simulink model "Actuator_testing"  (R2025b)
settings: Solver=VariableStepAuto  StartTime=0.0  StopTime=10.0  RelTol=1e-3
settings Model: Creator=Admin  LastModifiedBy=Admin

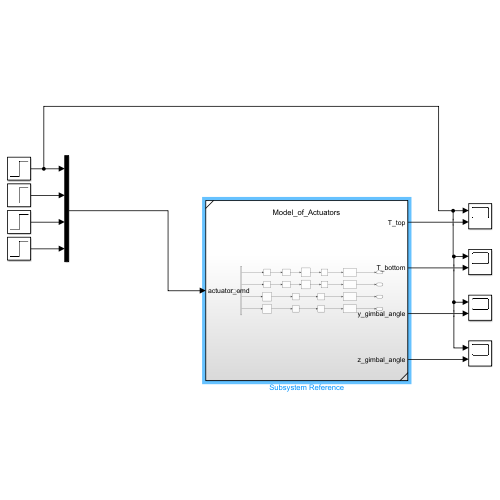
[thumbnail: Simulink's stored preview of the top-level diagram]
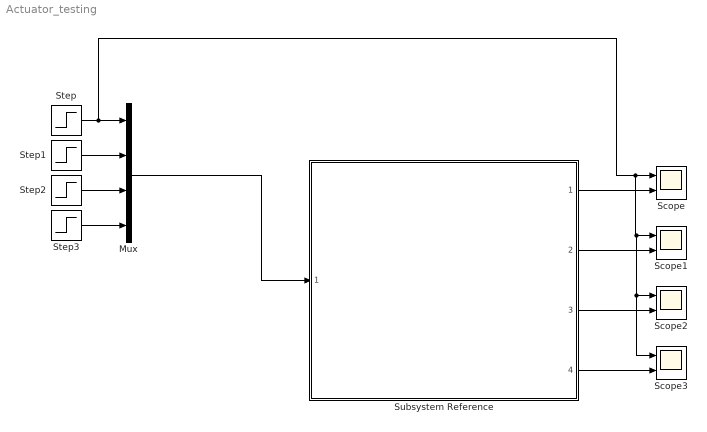
== system Actuator_testing ==
  Mux : Mux
  Scope{,1..3} (4 alike) : Scope  NumInputPorts=2
      Scope settings: ActiveDisplayYMinimum=-0.13072872674571806  ActiveDisplayYMaximum=1.1765585407114627
      Scope1 settings: ActiveDisplayYMinimum=-1  ActiveDisplayYMaximum=1
      Scope2 settings: ActiveDisplayYMinimum=-0.12499999999999997  ActiveDisplayYMaximum=1.125  DataLoggingVariableName=ScopeData2
      Scope3 settings: ActiveDisplayYMinimum=-0.12499999999999997  ActiveDisplayYMaximum=1.125  DataLoggingVariableName=ScopeData3
  Step{,1..3} (4 alike) : Step  SampleTime=0
  Subsystem Reference : Subsystem  ReferencedSubsystem=Model_of_Actuators
  wires:
  Step1/1 -> Mux/2
  Step/1 -> Scope3/1, Scope2/1, Scope1/1, Scope/1, Mux/1
  Step3/1 -> Mux/4
  Step2/1 -> Mux/3
  Mux/1 -> Subsystem Reference/1
  Subsystem Reference/1 -> Scope/2
  Subsystem Reference/2 -> Scope1/2
  Subsystem Reference/3 -> Scope2/2
  Subsystem Reference/4 -> Scope3/2
